simulink model "ADN"  (R2023b)
settings: Solver=ode1  StartTime=0.0  StopTime=1.5  FixedStep=Ts  RelTol=1e-3
undefined symbols (not defined in the file or in its folder): delta_E, delta_theta_deg, enable_breaker, fn, L_12, L_23, L_34, L_35, Lg, R_12, R_23, R_34, R_35, Rg, Tf, Ts, Un
libraries: spsLoadFlowBusLib x5, spsThreePhaseParallelRLCLoadLib x5, spsThreePhaseSeriesRLCBranchLib x5, ee_lib x3, GFL_Lib x2, spsSequenceAnalyzerLib x2, spsThreePhaseDynamicLoadLib x2, GFM_Lib x1, Source_Lib x1, spsPower3phInstantaneousLib x1, eeRmsMeasurement x1, spsThreePhaseSeriesRLCLoadLib x1
settings Model: Creator=Frederic_Colas  LastModifiedBy=pcstudentgele11
settings ModelReferenceCC: EnableRefExpFcnMdlSchedulingChecks=on
settings RTWCC: DLArmComputeVersion=19.05

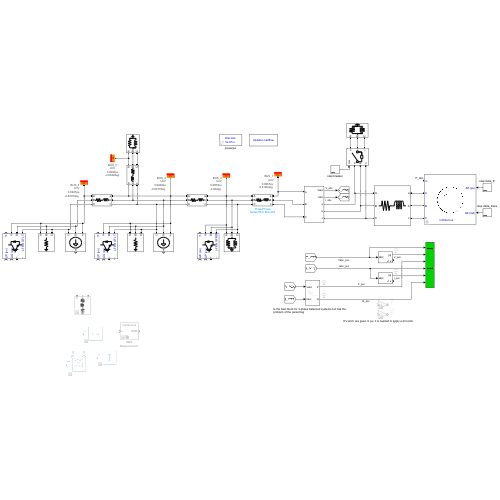
[thumbnail: Simulink's stored preview of the top-level diagram]
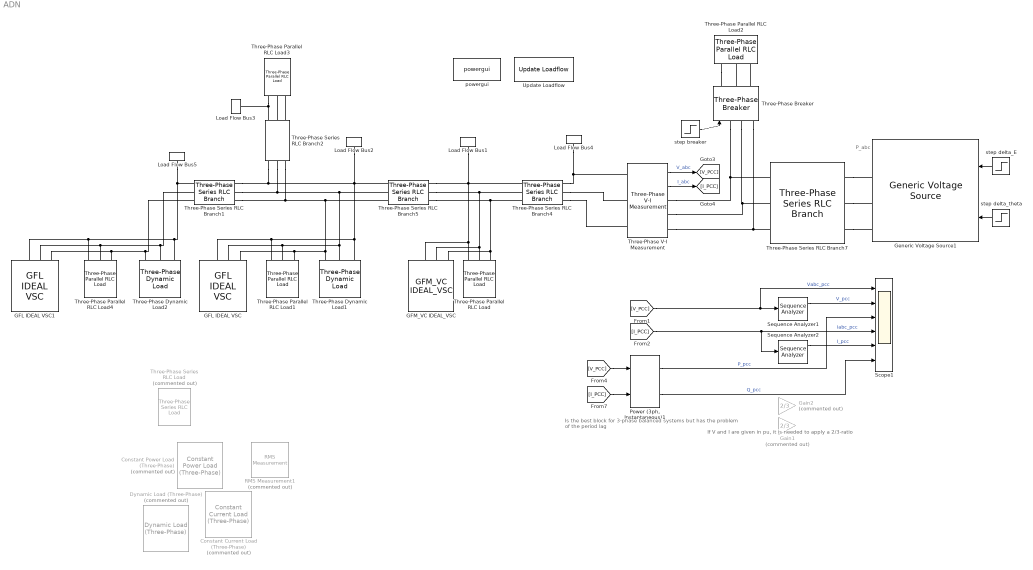
== system ADN ==
  note: P_abc
  note: Is the best block for 3-phase balanced systems but has the problem of the period lag
  note: If V and I are given in pu, it is needed to apply a 2/3-ratio
  Constant Current Load (Three-Phase) : ee_lib/Passive/Constant Current Load (Three-Phase)  Commented=on  consumed_current_rms=1 A  Vline_rms_min=10 V  enable_fault=simscape.enum.onoff.off  open_conductance=1e-4 S  fault_action=simscape.enum.assert.action.none  fault_trigger=ee.enum.faults.faultTrigger.temporal  t_fault=1 s  max_permissible_power=inf W  t_fail_on_power=1 s  faulted_open_circuit_specify=off  faulted_open_circuit_priority=None  faulted_open_circuit=0
      settings: InternalSimscapePortConfiguration="{\"Bottom\":[],\"Left\":[{\"id\":\"N\",\"label\":\"~\",\"type\":\"foundation.electrical.three_phase\"}],\"Right\":[],\"Top\":[]}"
  Constant Power Load (Three-Phase) : ee_lib/Passive/Constant Power Load (Three-Phase)  Commented=on  port_option=ee.enum.threePhasePort.composite  FRated=60 Hz  active_power=1 kW  reactive_power=0 A*kV  Vline_rms_min=100 V  tau=0.01 s  Vline_rms_ini=200 V  Vang_ini=0 deg  gmin=1e-6 S  enable_fault=simscape.enum.onoff.off  fault_action=simscape.enum.assert.action.none  t_fault=1 s  open_conductance=1e-4 S
      settings: InternalSimscapePortConfiguration="{\"Bottom\":[],\"Left\":[{\"id\":\"N\",\"label\":\"~\",\"type\":\"foundation.electrical.three_phase\"}],\"Right\":[],\"Top\":[]}"
  Dynamic Load (Three-Phase) : ee_lib/Passive/Dynamic Load (Three-Phase)  Commented=on  port_option=ee.enum.threePhasePort.composite  FRated=60 Hz  Vline_rms_min=100 V  tau=0.01 s  Vline_rms_ini=200 V  Vang_ini=0 deg  gmin=0 S  enable_fault=simscape.enum.onoff.off  fault_action=simscape.enum.assert.action.none  t_fault=1 s  open_conductance=1e-4 S
      settings: InternalSimscapePortConfiguration="{\"Bottom\":[],\"Left\":[{\"id\":\"N\",\"label\":\"~\",\"type\":\"foundation.electrical.three_phase\"}],\"Right\":[],\"Top\":[{\"id\":\"P\",\"label\":\"P\",\"type\":\"input\"},{\"id\":\"Q\",\"label\":\"Q\",\"type\":\"input\"}]}"
  GFL IDEAL VSC : GFL_Lib/GFL IDEAL VSC  fn=fn  Sn=Sn_GFL_3  Pn=Sn_GFL_3  Udcn=Vdc  Output_Delay=DelayGFL  Un1=Vnvsc  Un2=Un  m=1  Rt_pu=0.005  Lt_pu=0.15  Lm_pu=500  Rm_pu=500  DC_Link=Perfect DC Source  H_DC=inf  H_DC_sav=inf  wn_PLL=wpll_3  zeta_PLL=1  QV=Reactive Power Control  w_P=wp_3  w_V=wv_3  w_LPF=30  wn_i=wi_3  zeta_i=1  Kffi=on  Filtre_FF=on  w_ff=wff_3  Imax=1  Iqmax=0.3  K_FRT=0  Advanced=on  LFpopup=PQ  P0=0.5  Q0=4.5175e-18  V0=0.99483  Theta0=-0.83767
      settings: SourceProductName=VSC4SPS
  GFL IDEAL VSC1 : GFL_Lib/GFL IDEAL VSC  fn=fn  Sn=Sn_GFL_4  Pn=Sn_GFL_4  Udcn=Vdc  Output_Delay=DelayGFL  Un1=Vnvsc  Un2=Un  m=1  Rt_pu=0.005  Lt_pu=0.15  Lm_pu=500  Rm_pu=500  DC_Link=Perfect DC Source  H_DC=inf  H_DC_sav=inf  wn_PLL=wpll_4  zeta_PLL=1  QV=Reactive Power Control  w_P=wp_4  w_V=wv_4  w_LPF=30  wn_i=wi_4  zeta_i=1  Kffi=on  Filtre_FF=on  w_ff=wff_4  Imax=1  Iqmax=0.3  K_FRT=0  Advanced=on  LFpopup=PQ  P0=0.5  Q0=5.421e-18  V0=0.99471  Theta0=-0.83972
      settings: SourceProductName=VSC4SPS
  GFM_VC IDEAL_VSC : GFM_Lib/GFM_VC IDEAL_VSC  fn=fn  Sn=Sn_GFM_2  Pn=Sn_GFM_2  Udcn=Vdc  Output_Delay=DelayGFM  Un1=Vnvsc  Un2=Un  Rt_pu=0.005  Lt_pu=0.15  Lm_pu=500  Rm_pu=500  DC_Link=Perfect DC Source  H_DC=inf  H_DC_sav=40  wn_PLL=50  zeta_PLL=1  Val_Freq_Support=on  R_percent=8  dLc_pu=0  Rv=Rv_GFM_2  W_TVR=W_TVR  I_max_pu=1.2  wn_I_max=300  I_Max_TVI_pu=1.2  DX_DR=5  Advanced=on  gainpopup=With Inertia  wn_Inertia_Less=10  Param_Inertia=PI  H_GFo=H_2  zeta_GFo=ksi_2  LFpopup=PQ  P0=0.5  Q0=0  V0=0.99532  Theta0=-0.83
      settings: SourceProductName=VSC4SPS
  Gain1 : Gain  Commented=on  Gain=2/3
  Gain2 : Gain  Commented=on  Gain=2/3
  Generic Voltage Source1 : Source_Lib/Generic Voltage Source  SourceNature_str=INFINITE  fn=fn  Sn=Sng  Un=Un  H_s=5  DroopOnOff=on  R_percent=4  TN=1  TD=2  Time_Step=Ts  LFpopup=Swing  P0=0.043433  Q0=0.0066068  V0=1  Theta0=0
      settings: SourceProductName=VSC4SPS
  Load Flow Bus1 : spsLoadFlowBusLib/Load Flow Bus  LConnTagsString=a  Phases=single  Connectors=on one side  ID=BUS_2  Vbase=Un  Vref=1  Vangle=0  VLF=0.9953  VLFb=1  VLFc=1  angleLF=-0.83  angleLFb=0  angleLFc=0
  Load Flow Bus2 : spsLoadFlowBusLib/Load Flow Bus  LConnTagsString=a  Phases=single  Connectors=on one side  ID=BUS_3  Vbase=Un  Vref=1  Vangle=0  VLF=0.9948  VLFb=1  VLFc=1  angleLF=-0.8377  angleLFb=0  angleLFc=0
  Load Flow Bus3 : spsLoadFlowBusLib/Load Flow Bus  LConnTagsString=a  Phases=single  Connectors=on one side  ID=BUS_5  Vbase=Un  Vref=1  Vangle=0  VLF=0.9948  VLFb=1  VLFc=1  angleLF=-0.8382  angleLFb=0  angleLFc=0
  Load Flow Bus4 : spsLoadFlowBusLib/Load Flow Bus  LConnTagsString=a  Phases=single  Connectors=on one side  ID=BUS_1  Vbase=Un  Vref=1  Vangle=0  VLF=0.9965  VLFb=1  VLFc=1  angleLF=-0.8198  angleLFb=0  angleLFc=0
  Load Flow Bus5 : spsLoadFlowBusLib/Load Flow Bus  LConnTagsString=a  Phases=single  Connectors=on one side  ID=BUS_4  Vbase=Un  Vref=1  Vangle=0  VLF=0.9947  VLFb=1  VLFc=1  angleLF=-0.8397  angleLFb=0  angleLFc=0
  "Power (3ph, Instantaneous)1" : spsPower3phInstantaneousLib/Power (3ph, Instantaneous)
  RMS Measurement1 : eeRmsMeasurement/RMS Measurement  Commented=on  LabelModeActiveChoice=Total  F=60  SpecifyHarmonics=off  K=[0 1 2]  Ts=0
      settings: LibrarySourceBlock=|
      | ee_sl_lib/Measurements/RMS
      | Measurement
  Scope1 : Scope  NumInputPorts=6
  Sequence Analyzer1 : spsSequenceAnalyzerLib/Sequence Analyzer  Freq=50  n=1  seq=Positive  InInit=[327.251830, 0.953500]  Ts=0
  Sequence Analyzer2 : spsSequenceAnalyzerLib/Sequence Analyzer  Freq=50  n=1  seq=Positive  InInit=[10.185836, 0]  Ts=0
  Three-Phase Dynamic Load1 : spsThreePhaseDynamicLoadLib/Three-Phase Dynamic Load  NominalVoltage=[ Un fn ]  ActiveReactivePowers=[2000 5.96311e-14]  PositiveSequence=[0.99483 -0.837666]  ExternalControl=off  NpNq=[1.3 2]  TimeConstants="[0.02  0.08  0.02  0.05]"  MinimumVoltage=0.7  Tfilter=1e-4  LoadFlowParameters=[4,0,0,0,0]
      settings: LibrarySourceBlock=|
      | sps_lib/Passives/Three-Phase
      | Dynamic Load
  Three-Phase Dynamic Load2 : spsThreePhaseDynamicLoadLib/Three-Phase Dynamic Load  NominalVoltage=[ Un fn ]  ActiveReactivePowers=[1800 -5.42101e-15]  PositiveSequence=[0.994711 -0.839722]  ExternalControl=off  NpNq=[1 2]  TimeConstants="[0.05  0.1  0.04  0.11]"  MinimumVoltage=0.7  Tfilter=1e-4  LoadFlowParameters=[4,0,0,0,0]
      settings: LibrarySourceBlock=|
      | sps_lib/Passives/Three-Phase
      | Dynamic Load
  Three-Phase Parallel RLC Load : spsThreePhaseParallelRLCLoadLib/Three-Phase Parallel RLC Load  LConnTagsString=A|B|C  Configuration=Y (grounded)  NominalVoltage=Un  Vabc=[1e3 1e3 1e3]  Vabcp=[1e3 1e3 1e3]  NominalFrequency=fn  UnbalancedPower=off  ActivePower=3.5e3  InductivePower=0.5e3  CapacitivePower=0  Pabc=[10e3 9e3 11e3]  QLabc=[100 90 110]  QCabc=[100 90 110]  Pabcp=[10e3 9e3 11e3]  QLabcp=[100 90 110]  QCabcp=[100 90 110]  Measurements=None  LoadType=constant Z
  Three-Phase Parallel RLC Load1 : spsThreePhaseParallelRLCLoadLib/Three-Phase Parallel RLC Load  LConnTagsString=A|B|C  Configuration=Y (grounded)  NominalVoltage=Un  Vabc=[1e3 1e3 1e3]  Vabcp=[1e3 1e3 1e3]  NominalFrequency=fn  UnbalancedPower=off  ActivePower=1e3  InductivePower=0  CapacitivePower=0  Pabc=[10e3 9e3 11e3]  QLabc=[100 90 110]  QCabc=[100 90 110]  Pabcp=[10e3 9e3 11e3]  QLabcp=[100 90 110]  QCabcp=[100 90 110]  Measurements=None  LoadType=constant Z
  Three-Phase Parallel RLC Load2 : spsThreePhaseParallelRLCLoadLib/Three-Phase Parallel RLC Load  LConnTagsString=A|B|C  Configuration=Y (grounded)  NominalVoltage=Un  Vabc=[1e3 1e3 1e3]  Vabcp=[1e3 1e3 1e3]  NominalFrequency=fn  UnbalancedPower=off  ActivePower=P_fault  InductivePower=Q_fault  CapacitivePower=0  Pabc=[10e3 9e3 11e3]  QLabc=[100 90 110]  QCabc=[100 90 110]  Pabcp=[10e3 9e3 11e3]  QLabcp=[100 90 110]  QCabcp=[100 90 110]  Measurements=None  LoadType=constant Z
  Three-Phase Parallel RLC Load3 : spsThreePhaseParallelRLCLoadLib/Three-Phase Parallel RLC Load  LConnTagsString=A|B|C  Configuration=Y (grounded)  NominalVoltage=Un  Vabc=[1e3 1e3 1e3]  Vabcp=[1e3 1e3 1e3]  NominalFrequency=fn  UnbalancedPower=off  ActivePower=1.6e3  InductivePower=100  CapacitivePower=0  Pabc=[10e3 9e3 11e3]  QLabc=[100 90 110]  QCabc=[100 90 110]  Pabcp=[10e3 9e3 11e3]  QLabcp=[100 90 110]  QCabcp=[100 90 110]  Measurements=None  LoadType=constant Z
  Three-Phase Parallel RLC Load4 : spsThreePhaseParallelRLCLoadLib/Three-Phase Parallel RLC Load  LConnTagsString=A|B|C  Configuration=Y (grounded)  NominalVoltage=Un  Vabc=[1e3 1e3 1e3]  Vabcp=[1e3 1e3 1e3]  NominalFrequency=fn  UnbalancedPower=off  ActivePower=1e3  InductivePower=0  CapacitivePower=0  Pabc=[10e3 9e3 11e3]  QLabc=[100 90 110]  QCabc=[100 90 110]  Pabcp=[10e3 9e3 11e3]  QLabcp=[100 90 110]  QCabcp=[100 90 110]  Measurements=None  LoadType=constant Z
  Three-Phase Series RLC Branch1 : spsThreePhaseSeriesRLCBranchLib/Three-Phase Series RLC Branch  LConnTagsString=A|B|C  RConnTagsString=A|B|C  BranchType=RL  Resistance=R_34  Inductance=L_34  Capacitance=1e-6  Measurements=None
  Three-Phase Series RLC Branch2 : spsThreePhaseSeriesRLCBranchLib/Three-Phase Series RLC Branch  LConnTagsString=A|B|C  RConnTagsString=A|B|C  BranchType=RL  Resistance=R_35  Inductance=L_35  Capacitance=1e-6  Measurements=None
  Three-Phase Series RLC Branch4 : spsThreePhaseSeriesRLCBranchLib/Three-Phase Series RLC Branch  LConnTagsString=A|B|C  RConnTagsString=A|B|C  BranchType=RL  Resistance=R_12  Inductance=L_12  Capacitance=1e-6  Measurements=None
  Three-Phase Series RLC Branch5 : spsThreePhaseSeriesRLCBranchLib/Three-Phase Series RLC Branch  LConnTagsString=A|B|C  RConnTagsString=A|B|C  BranchType=RL  Resistance=R_23  Inductance=L_23  Capacitance=1e-6  Measurements=None
  Three-Phase Series RLC Branch7 : spsThreePhaseSeriesRLCBranchLib/Three-Phase Series RLC Branch  LConnTagsString=A|B|C  RConnTagsString=A|B|C  BranchType=RL  Resistance=Rg  Inductance=Lg  Capacitance=1e-6  Measurements=None
  Three-Phase Series RLC Load : spsThreePhaseSeriesRLCLoadLib/Three-Phase Series RLC Load  Commented=on  LConnTagsString=A|B|C  Configuration=Y (grounded)  NominalVoltage=1000  Vabc=[1e3 1e3 1e3]  Vabcp=[1e3 1e3 1e3]  NominalFrequency=60  UnbalancedPower=off  ActivePower=10e3  InductivePower=100  CapacitivePower=100  Pabc=[10e3 9e3 11e3]  QLabc=[100 90 110]  QCabc=[100 90 110]  Pabcp=[10e3 9e3 11e3]  QLabcp=[100 90 110]  QCabcp=[100 90 110]  Measurements=None  LoadType=constant Z
  Three-Phase V-I Measurement : spsThreePhaseVIMeasurementLib/Three-Phase V-I Measurement  VoltageMeasurement=phase-to-ground  SetLabelV=off  LabelV=Vabc  Vpu=off  VpuLL=off  CurrentMeasurement=yes  SetLabelI=off  LabelI=Iabc  Ipu=off  Pbase=Sn  Vbase=U1n  OutputType=Complex  PhasorSimulation=off  PSBequivalent=0
  Three-Phase Breaker : spsThreePhaseBreakerLib/Three-Phase Breaker  InitialState=open  SwitchA=on  SwitchB=on  SwitchC=on  SwitchTimes=t_breaker  External=on  BreakerResistance=0.01  SnubberResistance=1e6  SnubberCapacitance=inf  Measurements=None
  Update Loadflow : VSC_Lib/Update Loadflow  ShowInLibBrowser=on
      settings: SourceProductName=VSC4SPS
  powergui : spspowerguiLib/powergui  Priority=1  SimulationMode=Discrete  SampleTime=Ts  frequency=60  Iterations=50  frequencyindice=50  Pbase=100000  ErrMax=1e-6  UnitsV=kV  UnitsW=MW  buscounter=14  FunctionMessages=off  echomessages=off  EnableUseOfTLC=off  CurrentSourceSwitches=off  DisableSnubberDevices=off  DisableRonSwitches=off  DisableVfSwitches=off  DisplayEquations=off  AutomaticDiscreteSolvers=off  SolverType=Tustin/Backward Euler (TBE)  Interpol=off  ExternalGateDelay=off  methode=off  Ts=100  x0status=blocks  SPID=on  SwTol=0  HookPort=off  NonlinearTolerance=1e-4  nMaxIteration=100  ContinueOnMaxIteration=off  RestoreLinks=warning  ResistiveCurrentMeasurement=off  Frange=[0:2:500]  Ylog=off  Xlog=on  ShowGrid=off  save=off  variable=ZData  structure=0  ZoomFFT=off  StartTime=0.0  cycles=1  DisplayStyle=1  fundamental=60  FreqAxis=off  MaxFrequency=1000  frequencyindicesteady=1  RmsSteady=1  display=off
  step breaker : Step  Time=Tf  After=enable_breaker  SampleTime=0
  step delta_E : Step  Time=Tf  After=delta_E  SampleTime=0
  step delta_theta : Step  Time=Tf  After=delta_theta_deg*pi/180  SampleTime=0
  wires:
  Three-Phase V-I Measurement/2 -> [I_PCC]  "I_abc"
  Three-Phase V-I Measurement/1 -> [V_PCC]  "V_abc"
  [V_PCC] -> Scope1/1, Sequence Analyzer1/1  "Vabc_pcc"
  [V_PCC] -> "Power (3ph, Instantaneous)1"/1
  [I_PCC] -> Scope1/4, Sequence Analyzer2/1  "Iabc_pcc"
  "Power (3ph, Instantaneous)1"/2 -> Scope1/6  "Q_pcc"
  Sequence Analyzer2/1 -> Scope1/5  "I_pcc"
  Sequence Analyzer1/1 -> Scope1/2  "V_pcc"
  "Power (3ph, Instantaneous)1"/1 -> Scope1/3  "P_pcc"
  [I_PCC] -> "Power (3ph, Instantaneous)1"/2
  step breaker/1 -> Three-Phase Breaker/1
  step delta_E/1 -> Generic Voltage Source1/1
  step delta_theta/1 -> Generic Voltage Source1/2
  connections:
  Load Flow Bus4/LConn1 -- Three-Phase Series RLC Branch4/RConn1 -- Three-Phase V-I Measurement/LConn1
  Three-Phase Series RLC Branch7/RConn3 -- Generic Voltage Source1/RConn3
  Three-Phase Series RLC Branch7/RConn2 -- Generic Voltage Source1/RConn2
  Three-Phase Series RLC Branch7/RConn1 -- Generic Voltage Source1/RConn1
  Three-Phase V-I Measurement/RConn1 -- Three-Phase Breaker/LConn1 -- Three-Phase Series RLC Branch7/LConn1
  Three-Phase V-I Measurement/RConn2 -- Three-Phase Breaker/LConn2 -- Three-Phase Series RLC Branch7/LConn2
  Three-Phase V-I Measurement/RConn3 -- Three-Phase Series RLC Branch7/LConn3 -- Three-Phase Breaker/LConn3
  Three-Phase Parallel RLC Load/LConn1 -- Three-Phase Series RLC Branch5/RConn1 -- Three-Phase Series RLC Branch4/LConn1 -- Load Flow Bus1/LConn1 -- GFM_VC IDEAL_VSC/RConn1
  Three-Phase Parallel RLC Load/LConn2 -- Three-Phase Series RLC Branch5/RConn2 -- Three-Phase Series RLC Branch4/LConn2 -- GFM_VC IDEAL_VSC/RConn2
  Three-Phase Parallel RLC Load/LConn3 -- Three-Phase Series RLC Branch5/RConn3 -- Three-Phase Series RLC Branch4/LConn3 -- GFM_VC IDEAL_VSC/RConn3
  Three-Phase Series RLC Branch4/RConn2 -- Three-Phase V-I Measurement/LConn2
  Three-Phase Series RLC Branch4/RConn3 -- Three-Phase V-I Measurement/LConn3
  Three-Phase Dynamic Load1/LConn1 -- Three-Phase Series RLC Branch5/LConn1 -- Load Flow Bus2/LConn1 -- Three-Phase Series RLC Branch2/RConn1 -- Three-Phase Series RLC Branch1/RConn1 -- Three-Phase Parallel RLC Load1/LConn1 -- GFL IDEAL VSC/RConn1
  Three-Phase Dynamic Load1/LConn2 -- Three-Phase Series RLC Branch5/LConn2 -- Three-Phase Series RLC Branch2/RConn2 -- Three-Phase Series RLC Branch1/RConn2 -- Three-Phase Parallel RLC Load1/LConn2 -- GFL IDEAL VSC/RConn2
  Three-Phase Dynamic Load1/LConn3 -- Three-Phase Series RLC Branch5/LConn3 -- Three-Phase Series RLC Branch2/RConn3 -- Three-Phase Series RLC Branch1/RConn3 -- Three-Phase Parallel RLC Load1/LConn3 -- GFL IDEAL VSC/RConn3
  Three-Phase Parallel RLC Load3/LConn1 -- Three-Phase Series RLC Branch2/LConn1 -- Load Flow Bus3/LConn1
  Three-Phase Series RLC Branch2/LConn2 -- Three-Phase Parallel RLC Load3/LConn2
  Three-Phase Series RLC Branch2/LConn3 -- Three-Phase Parallel RLC Load3/LConn3
  Three-Phase Dynamic Load2/LConn3 -- Three-Phase Series RLC Branch1/LConn3 -- Three-Phase Parallel RLC Load4/LConn3 -- GFL IDEAL VSC1/RConn3
  Three-Phase Series RLC Branch1/LConn2 -- Three-Phase Dynamic Load2/LConn2 -- GFL IDEAL VSC1/RConn2 -- Three-Phase Parallel RLC Load4/LConn2
  Three-Phase Series RLC Branch1/LConn1 -- Load Flow Bus5/LConn1 -- Three-Phase Dynamic Load2/LConn1 -- GFL IDEAL VSC1/RConn1 -- Three-Phase Parallel RLC Load4/LConn1
  Three-Phase Breaker/RConn2 -- Three-Phase Parallel RLC Load2/LConn2
  Three-Phase Breaker/RConn3 -- Three-Phase Parallel RLC Load2/LConn3
  Three-Phase Parallel RLC Load2/LConn1 -- Three-Phase Breaker/RConn1
